simulink model "Y3Tiltrotor_sim3_IINDI"  (R2025a)
settings: Solver=ode4  StartTime=0.0  StopTime=70  FixedStep=uavParam.sampleTime  RelTol=1e-3
PreLoadFcn:
  | filepath  = fileparts(get_param(bdroot, 'FileName'))
  | cd(filepath);
InitFcn:
  | Init_sim_IINDI;
values from neighbouring files (symbols this model uses):
  a_HOD_p = 5    [Init_sim_IINDI.m]
  a_HOD_q = 1    [Init_sim_IINDI.m]
  a_HOD_r = 5    [Init_sim_IINDI.m]
  a_HOD_u = 30    [Init_sim_IINDI.m]
  a_HOD_v = 30    [Init_sim_IINDI.m]
  a_HOD_w = 30    [Init_sim_IINDI.m]
  control = struct    [Init_sim_IINDI.m]
  env = struct    [InitData.m]
  flightState = struct    [Init_sim_IINDI.m]
  FWSpeed0 = 15    [Init_sim_IINDI.m]
  k_lpf_p = 50    [Init_sim_IINDI.m]
  k_lpf_q = 80    [Init_sim_IINDI.m]
  k_lpf_r = 5    [Init_sim_IINDI.m]
  k_lpf_u = 10    [Init_sim_IINDI.m]
  k_lpf_v = 1    [Init_sim_IINDI.m]
  k_lpf_w = 50    [Init_sim_IINDI.m]
  k_p = 5    [Init_sim_IINDI.m]
  k_q = 20    [Init_sim_IINDI.m]
  k_r = 1.5    [Init_sim_IINDI.m]
  k_u = 0.5    [Init_sim_IINDI.m]
  k_v = 0.5    [Init_sim_IINDI.m]
  k_w = 2    [Init_sim_IINDI.m]
  l_p = 18    [Init_sim_IINDI.m]
  l_q = 6    [Init_sim_IINDI.m]
  l_r = 10    [Init_sim_IINDI.m]
  l_u = 45    [Init_sim_IINDI.m]
  l_v = 3    [Init_sim_IINDI.m]
  l_w = 15    [Init_sim_IINDI.m]
  lamda_p = 2    [Init_sim_IINDI.m]
  lamda_q = 2    [Init_sim_IINDI.m]
  lamda_r = 1    [Init_sim_IINDI.m]
  lamda_u = 5    [Init_sim_IINDI.m]
  lamda_v = 1    [Init_sim_IINDI.m]
  lamda_w = 3    [Init_sim_IINDI.m]
  uavParam = struct    [InitData.m]
undefined symbols (not defined in the file or in its folder): a_HOD, a_HOD_uvw, ControlSampleTime, F, Light, MIL, Newton, Raphson
libraries: slpidlib x30, SignalEditorBlockLib x13, simulink x6, aerolibtransform2 x3, sharedtransform x3, robotcorelib x3, matrix_library x3, aerolibasang x2, aerolibutil x2, aerolibwind2 x2, shared6dof x1, aerolibatmos2 x1
(part 8 of 8)

== matlab function Y3Tiltrotor_sim3_IINDI/Y3 Tiltrotor Aircraft Model/Subsystem/Aerodynamic Forces and Moments/Compute Body Frame Aerodynamic Forces and Moments/Wind frame F& M/Longitudinal Channel/Cm/Cm(alpha) ==
  data: Cm_alpha output; alpha input
function Cm_alpha = piecewise_Cm_alpha(alpha)

    c1 = 0.000219;
    c2 = -0.011442;
    c3 = 0.056866;
    c4 = -3.422369;
    c5 = -1.763366;
    c6 = -0.059447;
    c7 = 3.052526;
    c8 = 0.000256;
    c9 = -3.005585;
    c10 = -0.035985;
    c11 = -15.643618;

    Cm_alpha = zeros(size(alpha));

    idx_pos = alpha >= 0;
    if any(idx_pos)
        alpha_pos = alpha(idx_pos);
        Cm_alpha(idx_pos) = (1+tanh(c1*(18.4^2-alpha_pos.^2)))/(1+tanh(c1*18.4^2)).*(c2+c3*sin(c4*pi/180*alpha_pos))...
            +(1-(1+tanh(c1*(18.4^2-alpha_pos.^2)))/(1+tanh(c1*18.4^2))).*(c5*sin(c6*pi/180*alpha_pos+c7));
    end
    
    idx_neg = alpha < 0;
    if any(idx_neg)
        alpha_neg = alpha(idx_neg);
        Cm_alpha(idx_neg) = (1+tanh(c8*(15^2-alpha_neg.^2)))/(1+tanh(c8*15^2)).*(c2+c3*sin(c4*pi/180*alpha_neg))...
            +(1-(1+tanh(c8*(15^2-alpha_neg.^2)))/(1+tanh(c8*15^2))).*(c9*sin(c10*pi/180*alpha_neg+c11));
    end

end

== matlab function Y3Tiltrotor_sim3_IINDI/Y3 Tiltrotor Aircraft Model/Subsystem/Aerodynamic Forces and Moments/Compute Body Frame Aerodynamic Forces and Moments/Wind frame F& M/Lateral Channel/CY/CY(beta) ==
  data: CY_beta output; beta input
function CY_beta = fcn_CY_beta(beta)

    c1 = 65.424349;
    c2 = 41.5;
    c3 = 0.100430;
    c4 = -1.744107;
    c5 = 0.083409;
    c6 = 1.914772;
    c7 = -3.141796;

    CY_beta = (1+tanh(c1*(c2^2-beta.^2)))/(1+tanh(c1*c2^2)).*(c3*sin(c4*pi/180*beta))...
        + (1-(1+tanh(c1*(c2^2-beta.^2)))/(1+tanh(c1*c2^2))).*(c5*sin(c6*pi/180*beta+c7));

end

== matlab function Y3Tiltrotor_sim3_IINDI/Y3 Tiltrotor Aircraft Model/Subsystem/Aerodynamic Forces and Moments/Compute Body Frame Aerodynamic Forces and Moments/Wind frame F& M/Lateral Channel/Cl/Cl(beta) ==
  data: Cl1_beta output; beta input
function Cl1_beta = fcn_Cl1_beta(beta)

    c1 = 18.339628;
    c2 = 41.5;
    c3 = 0.035354;
    c4 = -1.788085;
    c5 = 0.035299;
    c6 = -1.515415;
    c7 = 0.001573;

    Cl1_beta = (1+tanh(c1*(c2^2-beta.^2)))/(1+tanh(c1*c2^2)).*(c3*sin(c4*pi/180*beta))...
        + (1-(1+tanh(c1*(c2^2-beta.^2)))/(1+tanh(c1*c2^2))).*(c5*sin(c6*pi/180*beta+c7));

end

== matlab function Y3Tiltrotor_sim3_IINDI/Y3 Tiltrotor Aircraft Model/Subsystem/Aerodynamic Forces and Moments/Compute Body Frame Aerodynamic Forces and Moments/Wind frame F& M/Lateral Channel/Cn/Cn(beta) ==
  data: Cn_beta output; beta input
function Cn_beta = fcn_Cn_beta(beta)

    c1 = 16.018126;
    c2 = 41.5;
    c3 = 0.045296;
    c4 = 0.918923;
    c5 = 0.028417;
    c6 = 1.203453;
    c7 = 6.274968;

    Cn_beta = (1+tanh(c1*(c2^2-beta.^2)))/(1+tanh(c1*c2^2)).*(c3*sin(c4*pi/180*beta))...
        + (1-(1+tanh(c1*(c2^2-beta.^2)))/(1+tanh(c1*c2^2))).*(c5*sin(c6*pi/180*beta+c7));

end

== matlab function Y3Tiltrotor_sim3_IINDI/Y3 Tiltrotor Aircraft Model/Subsystem/Aerodynamic Forces and Moments/Compute Body Frame Aerodynamic Forces and Moments/Wind frame F& M/Longitudinal Channel/Cm/Cm(delta_e) ==
  data: delta_e input; Cm_delta_e output
function Cm_delta_e = fcn_Cm_delta_e(delta_e)

    c1 = 0.000301;
    c2 = -1.724970;
    c3 = 0.142608;
    c4 = 0.109046;
    c5 = 0.694663;
    c6 = -2.968985;

    Cm_delta_e = (1+tanh(c1*(47.5^2-delta_e.^2)))/(1+tanh(c1*47.5^2)).*(c2*sin(c3*pi/180*delta_e))...
            +(1-(1+tanh(c1*(47.5^2-delta_e.^2)))/(1+tanh(c1*47.5^2))).*(c4*sin(c5*pi/180*delta_e+c6));

end

== matlab function Y3Tiltrotor_sim3_IINDI/Y3 Tiltrotor Aircraft Model/Subsystem/Aerodynamic Forces and Moments/Compute Body Frame Aerodynamic Forces and Moments/Wind frame F& M/Longitudinal Channel/CD/CD(delta_e) ==
  data: delta_e input; CD_delta_e output
function CD_delta_e = fcn_CD_delta_e(delta_e)

    c1 = 0.000707;
    c2 = 0.000057;
    c3 = 0.013601;
    c4 = 0.101850;
    c5 = 1.443831;
    c6 = 56.012704;
    c7 = 0.000024;
    c8 = 0.101300;
    c9 = -0.021731;
    c10 = -3.024408;
    c11 = 61.266062;

    CD_delta_e = zeros(size(delta_e));

    idx_pos = delta_e >= 0;
    if any(idx_pos)
        delta_e_pos = delta_e(idx_pos);
        CD_delta_e(idx_pos) = (1+tanh(c1*(47.4^2-delta_e_pos.^2)))/(1+tanh(c1*47.4^2)).*(c2*delta_e_pos.^2)...
            +(1-(1+tanh(c1*(47.4^2-delta_e_pos.^2)))/(1+tanh(c1*47.4^2))).*(c3+c4*sin(c5*pi/180*delta_e_pos+c6).^2);
    end

    idx_neg = delta_e < 0;
    if any(idx_neg)
        delta_e_neg = delta_e(idx_neg);
        CD_delta_e(idx_neg) = (1+tanh(c1*(47.4^2-delta_e_neg.^2)))/(1+tanh(c1*47.4^2)).*(c7*delta_e_neg.^2)...
            +(1-(1+tanh(c1*(47.4^2-delta_e_neg.^2)))/(1+tanh(c1*47.4^2))).*(c8+c9*sin(c10*pi/180*delta_e_neg+c11).^2);
    end
    
end
